simulink model "buildingClimateControl"  (R2025b)
settings: Solver=FixedStepDiscrete  StartTime=0.0  StopTime=10000  FixedStep=1  RelTol=1e-3  EnableMultiTasking=on
model workspace (MAT data in the model file):
  H_tol = 3
  T_tol = 2
libraries: simulink x2
settings Model: ExtModeAutoUpdateStatusClock=off  Creator=The MathWorks, Inc.  LastModifiedBy=The MathWorks, Inc.
settings SolverCC: AlgebraicLoopSolver=TrustRegion
settings DataIOCC: LimitDataPoints=on  SaveFormat=Array  ReturnWorkspaceOutputs=off
settings OptimizationCC: ReuseModelBlockBuffer=off  ExpressionDepthLimit=2147483647.0  InitFltsAndDblsToZero=on  EfficientMapNaN2IntZero=off  LifeSpan=inf
settings DebuggingCC: SaveWithParameterizedLinksMsg=none  UnderspecifiedInitializationDetection=Classic  MergeDetectMultiDrivingBlocksExec=none  SignalResolutionControl=TryResolveAllWithWarning  SolverPrmCheckMsg=warning  MultiTaskDSMMsg=warning  MultiTaskCondExecSysMsg=none  FcnCallInpInsideContextMsg=warning  UnconnectedInputMsg=warning  UnconnectedOutputMsg=warning  UnconnectedLineMsg=warning  StateNameClashWarn=warning  SFUnexpectedBacktrackingDiag=warning  SFNoUnconditionalDefaultTransitionDiag=warning  SFExecutionAtInitializationDiag=none  ArithmeticOperatorsInVariantConditions=warning
settings HardwareCC: ProdBitPerPointer=32.0  ProdBitPerSizeT=32.0  ProdBitPerPtrDiffT=32.0  ProdLargestAtomicFloat=None  ProdIntDivRoundTo=Undefined  ProdEndianess=Unspecified  ProdWordSize=32.0  ProdHWDeviceType=32-bit Generic
settings ModelReferenceCC: EnableRefExpFcnMdlSchedulingChecks=on  PropagateSignalLabelsOutOfModel=off
settings SFSimCC: SimUseLocalCustomCode=off  SimParseCustomCode=off  CustomCodeUndefinedFunction=UseInterfaceOnly
settings RTWCC: RTWUseLocalCustomCode=off  GPUComputeCapability=3.5  DLArmComputeVersion=19.05
settings CodeAppCC: StateflowObjectComments=on
settings GRTTargetCC: TargetFcnLib=ansi_tfl_tmw.mat  TargetLangStandard=C89/C90 (ANSI)  CombineOutputUpdateFcns=off  GRTInterface=on
settings ConfigComp: CovMetricSettings=dw  CovSaveCumulativeToWorkspaceVar=on  CovSaveSingleToWorkspaceVar=on  CovExternalEMLEnable=off  CovSFcnEnable=off

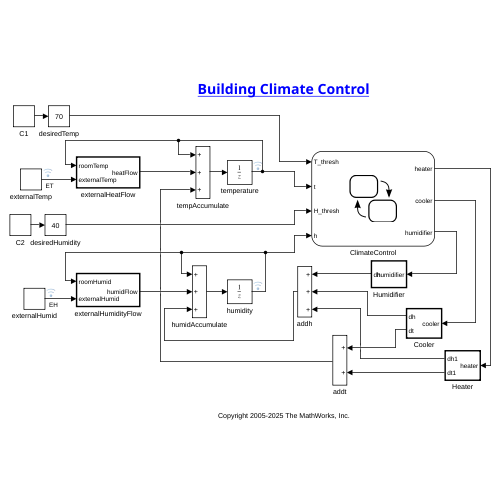
[thumbnail: Simulink's stored preview of the top-level diagram]
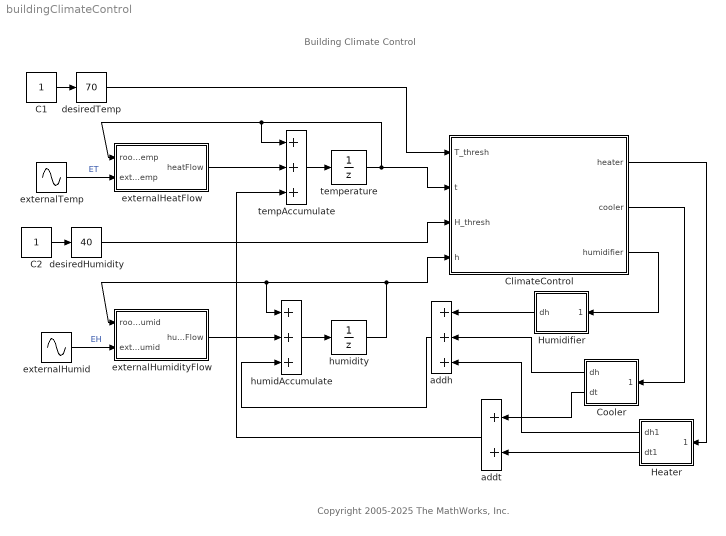
== system buildingClimateControl ==
  note: Copyright 2005-2025 The MathWorks, Inc.
  note: Building Climate Control
  C1 : Constant
  C2 : Constant
  ClimateControl : Stateflow chart  TreatAsAtomicUnit=on
  Cooler : Subsystem  TreatAsAtomicUnit=on
  Heater : Subsystem  TreatAsAtomicUnit=on
  Humidifier : Subsystem  TreatAsAtomicUnit=on
  addh : Sum  Inputs=+++
  addt : Sum
  desiredHumidity : simulink/Math Operations/Slider Gain  gain=40  low=30  high=60
  desiredTemp : simulink/Math Operations/Slider Gain  gain=70  low=50  high=90
  externalHeatFlow : Subsystem  TreatAsAtomicUnit=on
  externalHumid : Sin  Amplitude=10  Bias=40  Frequency=1/(24*60)  SampleTime=1
  externalHumidityFlow : Subsystem  TreatAsAtomicUnit=on
  externalTemp : Sin  Amplitude=10  Bias=70  Frequency=1/(24*60)  SampleTime=1
  humidAccumulate : Sum  Inputs=+++
  humidity : UnitDelay  InitialCondition=50  HasFrameUpgradeWarning=on
  tempAccumulate : Sum  Inputs=+++
  temperature : UnitDelay  InitialCondition=50  HasFrameUpgradeWarning=on
  wires:
  ClimateControl/3(humidifier) -> Humidifier/1(humidifier)
  temperature/1 -> ClimateControl/2(t), externalHeatFlow/1(roomTemp), tempAccumulate/1
  Cooler/1(dh) -> addh/2
  Heater/1(dh1) -> addh/3
  Cooler/2(dt) -> addt/1
  Heater/2(dt1) -> addt/2
  Humidifier/1(dh) -> addh/1
  addt/1 -> tempAccumulate/3
  ClimateControl/2(cooler) -> Cooler/1(cooler)
  ClimateControl/1(heater) -> Heater/1(heater)
  externalTemp/1 -> externalHeatFlow/2(externalTemp)  "ET"
  externalHumid/1 -> externalHumidityFlow/2(externalHumid)  "EH"
  externalHeatFlow/1(heatFlow) -> tempAccumulate/2
  tempAccumulate/1 -> temperature/1
  humidAccumulate/1 -> humidity/1
  humidity/1 -> ClimateControl/4(h), externalHumidityFlow/1(roomHumid), humidAccumulate/1
  externalHumidityFlow/1(humidFlow) -> humidAccumulate/2
  addh/1 -> humidAccumulate/3
  C1/1 -> desiredTemp/1
  desiredTemp/1 -> ClimateControl/1(T_thresh)
  C2/1 -> desiredHumidity/1
  desiredHumidity/1 -> ClimateControl/3(H_thresh)

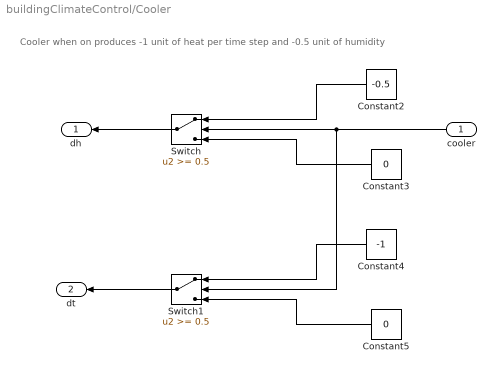
== system buildingClimateControl/Cooler ==
  note: Cooler when on produces -1 unit of heat per time step and -0.5 unit of humidity
  cooler : Inport
  Constant2 : Constant  Value=-0.5
  Constant3 : Constant  Value=0
  Constant4 : Constant  Value=-1
  Constant5 : Constant  Value=0
  Switch : Switch  Threshold=0.5  SaturateOnIntegerOverflow=off  InputSameDT=off
  Switch1 : Switch  Threshold=0.5  SaturateOnIntegerOverflow=off  InputSameDT=off
  dh : Outport  InitialOutput=0  VectorParamsAs1DForOutWhenUnconnected=off
  dt : Outport  Port=2  InitialOutput=0  VectorParamsAs1DForOutWhenUnconnected=off
  wires:
  cooler/1 -> Switch/2, Switch1/2
  Constant2/1 -> Switch/1
  Constant3/1 -> Switch/3
  Constant4/1 -> Switch1/1
  Constant5/1 -> Switch1/3
  Switch/1 -> dh/1
  Switch1/1 -> dt/1

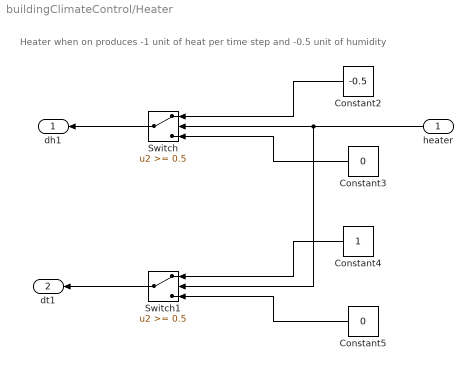
== system buildingClimateControl/Heater ==
  note: Heater when on produces -1 unit of heat per time step and -0.5 unit of humidity
  heater : Inport
  Constant2 : Constant  Value=-0.5
  Constant3 : Constant  Value=0
  Constant4 : Constant
  Constant5 : Constant  Value=0
  Switch : Switch  Threshold=0.5  SaturateOnIntegerOverflow=off  InputSameDT=off
  Switch1 : Switch  Threshold=0.5  SaturateOnIntegerOverflow=off  InputSameDT=off
  dh1 : Outport  InitialOutput=0  VectorParamsAs1DForOutWhenUnconnected=off
  dt1 : Outport  Port=2  InitialOutput=0  VectorParamsAs1DForOutWhenUnconnected=off
  wires:
  heater/1 -> Switch/2, Switch1/2
  Constant2/1 -> Switch/1
  Constant3/1 -> Switch/3
  Constant4/1 -> Switch1/1
  Constant5/1 -> Switch1/3
  Switch/1 -> dh1/1
  Switch1/1 -> dt1/1

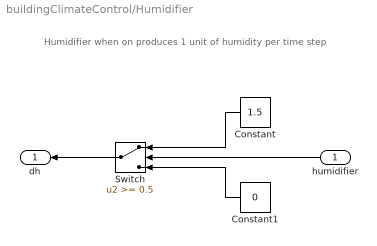
== system buildingClimateControl/Humidifier ==
  note: Humidifier when on produces 1 unit of humidity per time step
  humidifier : Inport
  Constant : Constant  Value=1.5
  Constant1 : Constant  Value=0
  Switch : Switch  Threshold=0.5  SaturateOnIntegerOverflow=off  InputSameDT=off
  dh : Outport  OutDataTypeStr=double  InitialOutput=0  VectorParamsAs1DForOutWhenUnconnected=off
  wires:
  humidifier/1 -> Switch/2
  Constant/1 -> Switch/1
  Constant1/1 -> Switch/3
  Switch/1 -> dh/1

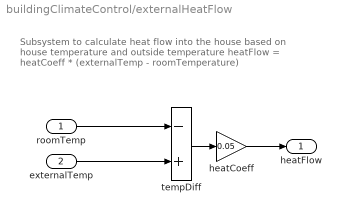
== system buildingClimateControl/externalHeatFlow ==
  note: Subsystem to calculate heat flow into the house based
      | on house temperature and outside temperature
      | heatFlow = heatCoeff * (externalTemp - roomTemperature)
  roomTemp : Inport
  externalTemp : Inport  Port=2
  heatCoeff : Gain  Gain=0.05
  tempDiff : Sum  Inputs=-+
  heatFlow : Outport  OutDataTypeStr=double  InitialOutput=0  VectorParamsAs1DForOutWhenUnconnected=off
  wires:
  tempDiff/1 -> heatCoeff/1
  heatCoeff/1 -> heatFlow/1
  roomTemp/1 -> tempDiff/1
  externalTemp/1 -> tempDiff/2

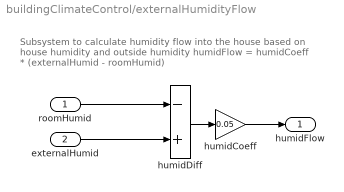
== system buildingClimateControl/externalHumidityFlow ==
  note: Subsystem to calculate humidity flow into the house based
      | on house humidity and outside humidity
      | humidFlow = humidCoeff * (externalHumid - roomHumid)
  roomHumid : Inport
  externalHumid : Inport  Port=2
  humidCoeff : Gain  Gain=0.05
  humidDiff : Sum  Inputs=-+
  humidFlow : Outport  OutDataTypeStr=double  InitialOutput=0  VectorParamsAs1DForOutWhenUnconnected=off
  wires:
  humidCoeff/1 -> humidFlow/1
  humidDiff/1 -> humidCoeff/1
  roomHumid/1 -> humidDiff/1
  externalHumid/1 -> humidDiff/2

== stateflow chart buildingClimateControl/ClimateControl ==
  state Temp [parallel]
    settings: executionOrder=1
    state HeatOn
      heater = 1;
      cooler = 0;
    state CoolOn
      cooler = 1;
      heater = 0;
    (default) -> HeatOn
    CoolOn -> HeatOn : [t <= T_thresh]
    HeatOn -> CoolOn : [t > T_thresh]
  state Humidity [parallel]
    settings: executionOrder=2
    state Off
      humidifier = 0;
    state On
      humidifier = 1;
    (default) -> Off
    On -> Off : [h >= H_thresh]
    Off -> On : [h <  H_thresh]
  data: heater output; T_thresh input; t input; H_thresh input; h input; cooler output; humidifier output
